simulink model "W13_ObserverBased"  (R2024b)
settings: Solver=ode45  StartTime=0.0  StopTime=t_end  MaxStep=0.001  RelTol=1e-3
PreLoadFcn:
  | % W13_ObserverBased 기본 파라미터 (모델을 열 때 자동 실행)
  | %
  | % [주의] setup_path 를 안 한 상태에서 모델만 열어도 돌아가야 합니다.
  | %        경로가 없으면 plant_dcmotor 를 못 찾으므로 아래처럼 숫자로 대신합니다.
  | if isempty(which('plant_dcmotor'))
  |     pp = struct('A', [0 1 0; 0 -10 1; 0 -0.02 -2], ...
  |                 'B', [0; 0; 2], 'C', [1 0 0], 'D', 0);
  | else
  |     [~, pp] = plant_dcmotor('position');
  | end
  | A_mat = pp.A;  B_mat = pp.B;  C_mat = pp.C;
  | L_obs = place(pp.A', pp.C', [-30 -34 -38])';
  | x0    = [0.5; 0; 0];
  | u_amp = 0;  noise_pwr = 0;  t_end = 1.0;
  | clear pp
libraries: simulink x1
settings Model: Creator=admin  LastModifiedBy=admin

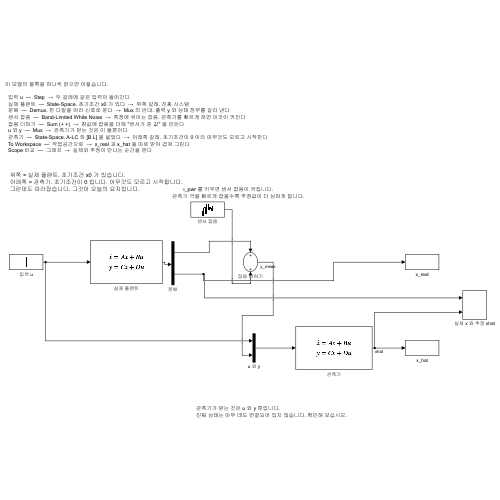
[thumbnail: Simulink's stored preview of the top-level diagram]
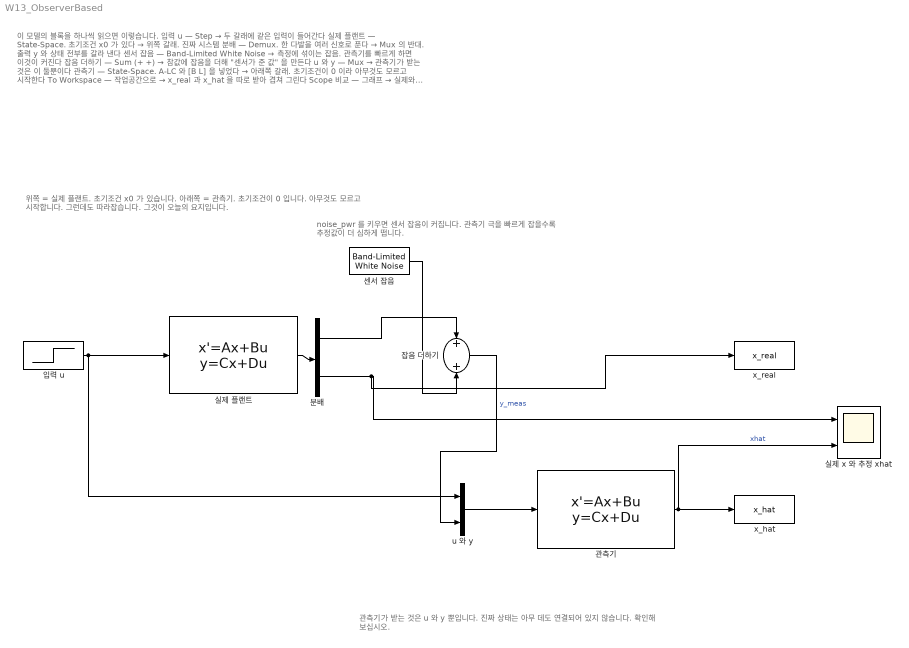
== system W13_ObserverBased ==
  note: 위쪽 = 실제 플랜트. 초기조건 x0 가 있습니다.
      | 아래쪽 = 관측기. 초기조건이 0 입니다. 아무것도 모르고 시작합니다.
      | 그런데도 따라잡습니다. 그것이 오늘의 요지입니다.
  note: 관측기가 받는 것은 u 와 y 뿐입니다.
      | 진짜 상태는 아무 데도 연결되어 있지 않습니다. 확인해 보십시오.
  note: noise_pwr 를 키우면 센서 잡음이 커집니다.
      | 관측기 극을 빠르게 잡을수록 추정값이 더 심하게 떱니다.
  note: 이 모델의 블록을 하나씩 읽으면 이렇습니다.
      |
      |   입력 u  —  Step  →  두 갈래에 같은 입력이 들어간다
      |   실제 플랜트  —  State-Space. 초기조건 x0 가 있다  →  위쪽 갈래. 진짜 시스템
      |   분배  —  Demux. 한 다발을 여러 신호로 푼다  →  Mux 의 반대. 출력 y 와 상태 전부를 갈라 낸다
      |   센서 잡음  —  Band-Limited White Noise  →  측정에 섞이는 잡음. 관측기를 빠르게 하면 이것이 커진다
      |   잡음 더하기  —  Sum (+ +)  →  참값에 잡음을 더해 "센서가 준 값" 을 만든다
      |   u 와 y  —  Mux  →  관측기가 받는 것은 이 둘뿐이다
      |   관측기  —  State-Space. A-LC 와 [B L] 을 넣었다  →  아래쪽 갈래. 초기조건이 0 이라 아무것도 모르고 시작한다
      |   To Workspace  —  작업공간으로  →  x_real 과 x_hat 을 따로 받아 겹쳐 그린다
      |   Scope 비교  —  그래프  →  실제와 추정이 만나는 순간을 본다
  u 와 y : Mux  Inputs=2
  x_hat : ToWorkspace  VariableName=x_hat  SaveFormat=Timeseries  SampleTime=-1
  x_real : ToWorkspace  VariableName=x_real  SaveFormat=Timeseries  SampleTime=-1
  관측기 : StateSpace  A=A_mat - L_obs*C_mat  B=[B_mat, L_obs]  C=eye(size(A_mat,1))  D=zeros(size(A_mat,1),2)  InitialCondition=zeros(size(A_mat,1),1)
  분배 : Demux  Outputs=[1 size(A_mat,1)]
  센서 잡음 : simulink/Sources/Band-Limited White Noise  Cov=noise_pwr  Ts=1e-4  seed=23341
  실제 x 와 추정 xhat : Scope  NumInputPorts=2
  실제 플랜트 : StateSpace  A=A_mat  B=B_mat  C=[C_mat; eye(size(A_mat,1))]  D=zeros(size(A_mat,1)+1, 1)  InitialCondition=x0
  입력 u : Step  Time=0  After=u_amp  SampleTime=0
  잡음 더하기 : Sum
  wires:
  입력 u/1 -> 실제 플랜트/1, u 와 y/1
  실제 플랜트/1 -> 분배/1
  분배/1 -> 잡음 더하기/1
  센서 잡음/1 -> 잡음 더하기/2
  분배/2 -> x_real/1, 실제 x 와 추정 xhat/1
  잡음 더하기/1 -> u 와 y/2  "y_meas"
  u 와 y/1 -> 관측기/1
  관측기/1 -> x_hat/1, 실제 x 와 추정 xhat/2  "xhat"
